simulink model "AGV_IFOC_BLOCKS"  (R2025a)
settings: Solver=ode4  StartTime=0.0  StopTime=t_stop_agv  FixedStep=h_step_agv  RelTol=1e-3
InitFcn:
  | addpath(fileparts(get_param('AGV_IFOC_BLOCKS','FileName'))); bm_drive = 'IFOC'; bm_model = 'AGV_IFOC_BLOCKS'; block_model_params;
values from neighbouring files (symbols this model uses):
  agv_fault_side_default = a.fault_side    [block_model_params.m]
  agv_fault_type_default = a.fault_type    [block_model_params.m]
  Bm = m.B    [block_model_params.m]
  Crr = a.Crr    [block_model_params.m]
  Esw = P.inv.Esw    [block_model_params.m]
  eta_g = a.eta_g    [block_model_params.m]
  flux_mode_default = c.flux_mode    [block_model_params.m]
  G_gear = a.G    [block_model_params.m]
  h_step_agv = 25e-6    (= 2.5e-05)    [block_model_params.m]
  Iref_sw = P.inv.Iref    [block_model_params.m]
  Jm = m.J    [block_model_params.m]
  ke = m.ke    [block_model_params.m]
  kh = m.kh    [block_model_params.m]
  Ki_i = c.Ki_i    [block_model_params.m]
  Ko = c.Ko    [block_model_params.m]
  Kp_i = c.Kp_i    [block_model_params.m]
  Kp_w = c.Kp_w    [block_model_params.m]
  L_look = a.L_look    [block_model_params.m]
  Llr = m.Llr    [block_model_params.m]
  Lls = m.Lls    [block_model_params.m]
  Lm0 = m.Lm0    [block_model_params.m]
  Lm_rated = m.Lm_rated    [block_model_params.m]
  lut_an = P.lut.psi    [block_model_params.m]
  lut_ml = bm_P.lut.psi; end    [block_model_params.m]
  lut_T = P.lut.T(:)'    [block_model_params.m]
  lut_w = P.lut.w(:)'    [block_model_params.m]
  Lx = a.Lx    [block_model_params.m]
  Ly = a.Ly    [block_model_params.m]
  m_payload = a.m_payload    [block_model_params.m]
  m_robot = a.m_robot    [block_model_params.m]
  mlp_b1 = double(bm_M.b1(:))    [block_model_params.m]
  mlp_b2 = double(bm_M.b2)    [block_model_params.m]
  mlp_W1 = double(bm_M.W1)    [block_model_params.m]
  mlp_W2 = double(bm_M.W2(:)')    [block_model_params.m]
  mlp_x_mu = double(bm_M.x_mu(:))    [block_model_params.m]
  mlp_x_sd = double(bm_M.x_sd(:))    [block_model_params.m]
  mlp_y_mu = double(bm_M.y_mu)    [block_model_params.m]
  mlp_y_sd = double(bm_M.y_sd)    [block_model_params.m]
  mras_Ki = c.mras_Ki    [block_model_params.m]
  mras_Kp = c.mras_Kp    [block_model_params.m]
  mras_wc = c.mras_wc    [block_model_params.m]
  NT_agv = max(1, round(Ts/h_step_agv))    [block_model_params.m]
  pp = m.p    [block_model_params.m]
  psi_k = m.psi_k    [block_model_params.m]
  r_wheel = a.r_wheel    [block_model_params.m]
  rce = P.inv.rce    [block_model_params.m]
  Rr = m.Rr    [block_model_params.m]
  Rs = m.Rs    [block_model_params.m]
  s32 = sqrt(3)/2    [block_model_params.m]
  sat_a = m.sat_a    [block_model_params.m]
  sat_b = m.sat_b    [block_model_params.m]
  sat_on = m.sat_on    [block_model_params.m]
  Te_max = c.Te_max    [block_model_params.m]
  Ts = P.ctrl.Ts    [block_log_to_thesis.m]    (also in block_model_params.m = c.Ts)
  twopi = 2*pi    (= 6.28318530718)    [block_model_params.m]
  Vce0 = P.inv.Vce0    [block_model_params.m]
  Vdc = P.inv.Vdc    [block_model_params.m]
  Vref_sw = P.inv.Vref    [block_model_params.m]
  W_track = a.W_track    [block_model_params.m]
(part 2 of 4)

== system AGV_IFOC_BLOCKS/Right wheel drive/Controller ==
  ia_m : Inport
  ib_m : Inport  Port=2
  ic_m : Inport  Port=3
  w_m : Inport  Port=4
  w_ref : Inport  Port=5
  flux_sel : Inport  Port=6
  lut_sel : Inport  Port=7
  speed_mode : Inport  Port=8
  Applied voltage and current observer : Subsystem
  Current reconstruction : Subsystem
  Fault detection and isolation : Subsystem
  Flux reference : Subsystem
  IFOC current control and SVPWM : Subsystem
  MRAS speed estimator : Subsystem
  Model inductances : Subsystem
  Speed controller : Subsystem
  Te_est not used in IFOC : Constant  Value=0
  ia_m sample : ZeroOrderHold  SampleTime=Ts
  ib_m sample : ZeroOrderHold  SampleTime=Ts
  ic_m sample : ZeroOrderHold  SampleTime=Ts
  w_m sample : ZeroOrderHold  SampleTime=Ts
  w_ref sample : ZeroOrderHold  SampleTime=Ts
  da out : Outport
  db out : Outport  Port=2
  dc out : Outport  Port=3
  neutral out : Outport  Port=4
  w_u out : Outport  Port=5
  w_est out : Outport  Port=6
  Te_ref out : Outport  Port=7
  psi_ref out : Outport  Port=8
  psi_est out : Outport  Port=9
  Te_est out : Outport  Port=10
  f_speed out : Outport  Port=11
  f_cur out : Outport  Port=12
  f_open out : Outport  Port=13
  wires:
  ia_m/1 -> ia_m sample/1
  ib_m/1 -> ib_m sample/1
  ic_m/1 -> ic_m sample/1
  w_m/1 -> w_m sample/1
  w_ref/1 -> w_ref sample/1
  Flux reference/3(psi_ref_p out) -> Model inductances/1(psi_ref_p)
  ia_m sample/1 -> Current reconstruction/1(ia_m), Fault detection and isolation/2(ia_m)
  ib_m sample/1 -> Current reconstruction/2(ib_m), Fault detection and isolation/3(ib_m), Applied voltage and current observer/4(ib_m)
  ic_m sample/1 -> Current reconstruction/3(ic_m), Fault detection and isolation/4(ic_m)
  Fault detection and isolation/8(f_cur_p out) -> Current reconstruction/4(f_cur_p)
  Fault detection and isolation/9(neutral_p out) -> Current reconstruction/5(neutral_p)
  Applied voltage and current observer/3(obs1_p out) -> Current reconstruction/6(obs1_p)
  Applied voltage and current observer/4(obs3_p out) -> Current reconstruction/7(obs3_p)
  Model inductances/1(Lm_c out) -> Current reconstruction/8(Lm_c), MRAS speed estimator/7(Lm_c), IFOC current control and SVPWM/8(Lm_c), Applied voltage and current observer/6(Lm_c)
  Model inductances/3(Lr_c out) -> Current reconstruction/9(Lr_c), MRAS speed estimator/8(Lr_c), IFOC current control and SVPWM/9(Lr_c), Applied voltage and current observer/8(Lr_c)
  Model inductances/6(D_c out) -> Current reconstruction/10(D_c), Applied voltage and current observer/9(D_c)
  Current reconstruction/1(i_alpha out) -> MRAS speed estimator/1(i_alpha), IFOC current control and SVPWM/1(i_alpha)
  Current reconstruction/2(i_beta out) -> MRAS speed estimator/2(i_beta), IFOC current control and SVPWM/2(i_beta)
  Current reconstruction/4(i_alpha_p out) -> MRAS speed estimator/3(i_alpha_p)
  Current reconstruction/5(i_beta_p out) -> MRAS speed estimator/4(i_beta_p)
  Applied voltage and current observer/1(va_app_p out) -> MRAS speed estimator/5(va_app_p)
  Applied voltage and current observer/2(vb_app_p out) -> MRAS speed estimator/6(vb_app_p)
  Model inductances/4(sLs_c out) -> MRAS speed estimator/9(sLs_c), IFOC current control and SVPWM/10(sLs_c)
  Model inductances/5(tr_c out) -> MRAS speed estimator/10(tr_c), IFOC current control and SVPWM/11(tr_c)
  w_ref sample/1 -> MRAS speed estimator/11(w_ref), Fault detection and isolation/5(w_ref), Speed controller/1(w_ref)
  w_m sample/1 -> MRAS speed estimator/12(w_m), Fault detection and isolation/1(w_m)
  Fault detection and isolation/7(f_speed_p out) -> MRAS speed estimator/13(f_speed_p)
  Flux reference/4(trans_t_p out) -> MRAS speed estimator/14(trans_t_p)
  Flux reference/5(dpsi_rate_p out) -> MRAS speed estimator/15(dpsi_p)
  Speed controller/3(Te_ref_p out) -> MRAS speed estimator/16(Te_ref_p)
  Fault detection and isolation/10(Te_lim_p out) -> MRAS speed estimator/17(Te_lim_p)
  MRAS speed estimator/1(w_est out) -> Fault detection and isolation/6(w_est), w_est out/1
  MRAS speed estimator/2(mras_ok out) -> Fault detection and isolation/7(mras_ok)
  Current reconstruction/3(ia_hat out) -> Fault detection and isolation/8(ia_hat)
  Fault detection and isolation/6(w_u out) -> Speed controller/2(w_u), Flux reference/3(w_u), IFOC current control and SVPWM/6(w_u), Applied voltage and current observer/5(w_u), w_u out/1
  Fault detection and isolation/5(Te_lim out) -> Speed controller/3(Te_lim)
  speed_mode/1 -> Speed controller/4(mode)
  Speed controller/2(e_w out) -> Flux reference/1(e_w)
  Speed controller/1(Te_ref out) -> Flux reference/2(Te_ref), IFOC current control and SVPWM/5(Te_ref), Te_ref out/1
  flux_sel/1 -> Flux reference/4(flux_sel)
  lut_sel/1 -> Flux reference/5(lut_sel)
  Flux reference/1(psi_ref out) -> IFOC current control and SVPWM/3(psi_ref), psi_ref out/1
  Flux reference/2(dpsi_rate out) -> IFOC current control and SVPWM/4(dpsi_rate)
  Fault detection and isolation/4(neutral out) -> IFOC current control and SVPWM/7(neutral), neutral out/1
  Te_est not used in IFOC/1 -> Te_est out/1
  IFOC current control and SVPWM/1(da out) -> Applied voltage and current observer/1(da), da out/1
  IFOC current control and SVPWM/2(db out) -> Applied voltage and current observer/2(db), db out/1
  IFOC current control and SVPWM/3(dc out) -> Applied voltage and current observer/3(dc), dc out/1
  Model inductances/2(Ls_c out) -> Applied voltage and current observer/7(Ls_c)
  IFOC current control and SVPWM/4(psir_est out) -> psi_est out/1
  Fault detection and isolation/1(f_speed out) -> f_speed out/1
  Fault detection and isolation/2(f_cur out) -> f_cur out/1
  Fault detection and isolation/3(f_open out) -> f_open out/1

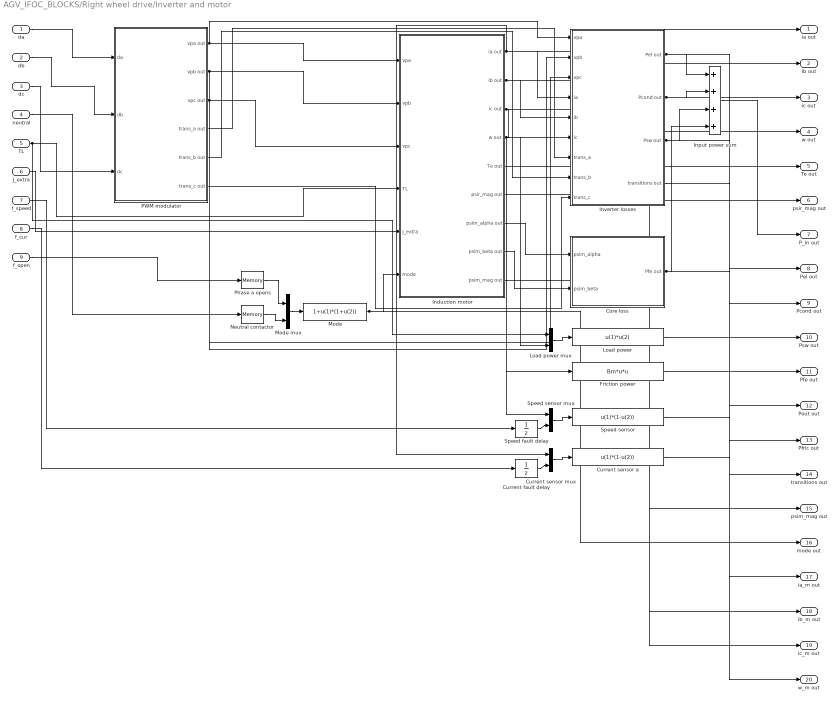
== system AGV_IFOC_BLOCKS/Right wheel drive/Inverter and motor ==
  da : Inport
  db : Inport  Port=2
  dc : Inport  Port=3
  neutral : Inport  Port=4
  TL : Inport  Port=5
  J_extra : Inport  Port=6
  f_speed : Inport  Port=7
  f_cur : Inport  Port=8
  f_open : Inport  Port=9
  Core loss : Subsystem
  Current fault delay : UnitDelay  SampleTime=Ts  HasFrameUpgradeWarning=on
  Current sensor a : Fcn  Expr=u(1)*(1-u(2))
  Current sensor mux : Mux  Inputs=2
  Friction power : Fcn  Expr=Bm*u*u
  Induction motor : Subsystem
  Input power sum : Sum  Inputs=++++
  Inverter losses : Subsystem
  Load power : Fcn  Expr=u(1)*u(2)
  Load power mux : Mux  Inputs=2
  Mode : Fcn  Expr=1+u(1)*(1+u(2))
  Mode mux : Mux  Inputs=2
  Neutral contactor : Memory
  PWM modulator : Subsystem
  Phase a opens : Memory
  Speed fault delay : UnitDelay  SampleTime=Ts  HasFrameUpgradeWarning=on
  Speed sensor : Fcn  Expr=u(1)*(1-u(2))
  Speed sensor mux : Mux  Inputs=2
  ia out : Outport
  ib out : Outport  Port=2
  ic out : Outport  Port=3
  w out : Outport  Port=4
  Te out : Outport  Port=5
  psir_mag out : Outport  Port=6
  P_in out : Outport  Port=7
  Pel out : Outport  Port=8
  Pcond out : Outport  Port=9
  Psw out : Outport  Port=10
  Pfe out : Outport  Port=11
  Pout out : Outport  Port=12
  Pfric out : Outport  Port=13
  transitions out : Outport  Port=14
  psim_mag out : Outport  Port=15
  mode out : Outport  Port=16
  ia_m out : Outport  Port=17
  ib_m out : Outport  Port=18
  ic_m out : Outport  Port=19
  w_m out : Outport  Port=20
  wires:
  neutral/1 -> Neutral contactor/1
  f_open/1 -> Phase a opens/1
  Phase a opens/1 -> Mode mux/1
  Neutral contactor/1 -> Mode mux/2
  Mode mux/1 -> Mode/1
  da/1 -> PWM modulator/1(da)
  db/1 -> PWM modulator/2(db)
  dc/1 -> PWM modulator/3(dc)
  PWM modulator/1(vpa out) -> Induction motor/1(vpa), Inverter losses/1(vpa)
  PWM modulator/2(vpb out) -> Induction motor/2(vpb), Inverter losses/2(vpb)
  PWM modulator/3(vpc out) -> Induction motor/3(vpc), Inverter losses/3(vpc)
  TL/1 -> Induction motor/4(TL), Load power mux/1
  J_extra/1 -> Induction motor/5(J_extra)
  Mode/1 -> Induction motor/6(mode), mode out/1
  Induction motor/1(ia out) -> Inverter losses/4(ia), Current sensor mux/1, ia out/1
  PWM modulator/4(trans_a out) -> Inverter losses/7(trans_a)
  Induction motor/2(ib out) -> Inverter losses/5(ib), ib out/1, ib_m out/1
  PWM modulator/5(trans_b out) -> Inverter losses/8(trans_b)
  Induction motor/3(ic out) -> Inverter losses/6(ic), ic out/1, ic_m out/1
  PWM modulator/6(trans_c out) -> Inverter losses/9(trans_c)
  Induction motor/7(psim_alpha out) -> Core loss/1(psim_alpha)
  Induction motor/8(psim_beta out) -> Core loss/2(psim_beta)
  Induction motor/4(w out) -> Load power mux/2, Friction power/1, Speed sensor mux/1, w out/1
  Load power mux/1 -> Load power/1
  Inverter losses/1(Pel out) -> Input power sum/1, Pel out/1
  Inverter losses/2(Pcond out) -> Input power sum/2, Pcond out/1
  Inverter losses/3(Psw out) -> Input power sum/3, Psw out/1
  Core loss/1(Pfe out) -> Input power sum/4, Pfe out/1
  f_speed/1 -> Speed fault delay/1
  f_cur/1 -> Current fault delay/1
  Speed fault delay/1 -> Speed sensor mux/2
  Speed sensor mux/1 -> Speed sensor/1
  Current fault delay/1 -> Current sensor mux/2
  Current sensor mux/1 -> Current sensor a/1
  Induction motor/5(Te out) -> Te out/1
  Induction motor/6(psir_mag out) -> psir_mag out/1
  Input power sum/1 -> P_in out/1
  Load power/1 -> Pout out/1
  Friction power/1 -> Pfric out/1
  Inverter losses/4(transitions out) -> transitions out/1
  Induction motor/9(psim_mag out) -> psim_mag out/1
  Current sensor a/1 -> ia_m out/1
  Speed sensor/1 -> w_m out/1

== system AGV_IFOC_BLOCKS/Left wheel drive/Controller/Applied voltage and current observer ==
  da : Inport
  db : Inport  Port=2
  dc : Inport  Port=3
  ib_m : Inport  Port=4
  w_u : Inport  Port=5
  Lm_c : Inport  Port=6
  Ls_c : Inport  Port=7
  Lr_c : Inport  Port=8
  D_c : Inport  Port=9
  ib error : Fcn  Expr=u(1)-(-0.5*u(2)+s32*u(3))
  ib error in : Mux  Inputs=3
  obs ir_alpha : Fcn  Expr=(u(6)*u(3)-u(5)*u(1))/u(8)
  obs ir_alpha in : Mux  Inputs=8
  obs ir_beta : Fcn  Expr=(u(6)*u(4)-u(5)*u(2))/u(8)
  obs ir_beta in : Mux  Inputs=8
  obs is_alpha : Fcn  Expr=(u(7)*u(1)-u(5)*u(3))/u(8)
  obs is_alpha in : Mux  Inputs=8
  obs is_beta : Fcn  Expr=(u(7)*u(2)-u(5)*u(4))/u(8)
  obs is_beta in : Mux  Inputs=8
  obs1 : Fcn  Expr=u(1)+Ts*(u(2)-Rs*u(3)+Ko*(-0.5)*u(4))
  obs1 in : Mux
  obs1(k-1) : UnitDelay  SampleTime=Ts  HasFrameUpgradeWarning=on
  obs2 : Fcn  Expr=u(1)+Ts*(u(2)-Rs*u(3)+Ko*s32*u(4))
  obs2 in : Mux
  obs2(k-1) : UnitDelay  SampleTime=Ts  HasFrameUpgradeWarning=on
  obs3 : Fcn  Expr=u(1)+Ts*(-Rr*u(3)-pp*u(4)*u(2))
  obs3 in : Mux
  obs3(k-1) : UnitDelay  SampleTime=Ts  HasFrameUpgradeWarning=on
  obs4 : Fcn  Expr=u(2)+Ts*(-Rr*u(3)+pp*u(4)*u(1))
  obs4 in : Mux
  obs4(k-1) : UnitDelay  SampleTime=Ts  HasFrameUpgradeWarning=on
  va_app : Fcn  Expr=(2/3)*((u(1)-0.5)*Vdc-0.5*((u(2)-0.5)*Vdc+(u(3)-0.5)*Vdc))
  va_app in : Mux  Inputs=3
  va_app(k-1) : UnitDelay  SampleTime=Ts  HasFrameUpgradeWarning=on
  vb_app : Fcn  Expr=((u(1)-0.5)*Vdc-(u(2)-0.5)*Vdc)/sqrt(3)
  vb_app in : Mux  Inputs=2
  vb_app(k-1) : UnitDelay  SampleTime=Ts  HasFrameUpgradeWarning=on
  va_app_p out : Outport
  vb_app_p out : Outport  Port=2
  obs1_p out : Outport  Port=3
  obs3_p out : Outport  Port=4
  wires:
  da/1 -> va_app in/1
  db/1 -> va_app in/2, vb_app in/1
  dc/1 -> va_app in/3, vb_app in/2
  va_app in/1 -> va_app/1
  va_app/1 -> va_app(k-1)/1, obs1 in/2
  vb_app in/1 -> vb_app/1
  vb_app/1 -> vb_app(k-1)/1, obs2 in/2
  obs1(k-1)/1 -> obs is_alpha in/1, obs is_beta in/1, obs ir_alpha in/1, obs ir_beta in/1, obs1 in/1, obs1_p out/1
  obs2(k-1)/1 -> obs is_alpha in/2, obs is_beta in/2, obs ir_alpha in/2, obs ir_beta in/2, obs2 in/1
  obs3(k-1)/1 -> obs is_alpha in/3, obs is_beta in/3, obs ir_alpha in/3, obs ir_beta in/3, obs3 in/1, obs4 in/1, obs3_p out/1
  obs4(k-1)/1 -> obs is_alpha in/4, obs is_beta in/4, obs ir_alpha in/4, obs ir_beta in/4, obs3 in/2, obs4 in/2
  Lm_c/1 -> obs is_alpha in/5, obs is_beta in/5, obs ir_alpha in/5, obs ir_beta in/5
  Ls_c/1 -> obs is_alpha in/6, obs is_beta in/6, obs ir_alpha in/6, obs ir_beta in/6
  Lr_c/1 -> obs is_alpha in/7, obs is_beta in/7, obs ir_alpha in/7, obs ir_beta in/7
  D_c/1 -> obs is_alpha in/8, obs is_beta in/8, obs ir_alpha in/8, obs ir_beta in/8
  obs is_alpha in/1 -> obs is_alpha/1
  obs is_beta in/1 -> obs is_beta/1
  obs ir_alpha in/1 -> obs ir_alpha/1
  obs ir_beta in/1 -> obs ir_beta/1
  ib_m/1 -> ib error in/1
  obs is_alpha/1 -> ib error in/2, obs1 in/3
  obs is_beta/1 -> ib error in/3, obs2 in/3
  ib error in/1 -> ib error/1
  ib error/1 -> obs1 in/4, obs2 in/4
  obs1 in/1 -> obs1/1
  obs1/1 -> obs1(k-1)/1
  obs2 in/1 -> obs2/1
  obs2/1 -> obs2(k-1)/1
  obs ir_alpha/1 -> obs3 in/3
  w_u/1 -> obs3 in/4, obs4 in/4
  obs3 in/1 -> obs3/1
  obs3/1 -> obs3(k-1)/1
  obs ir_beta/1 -> obs4 in/3
  obs4 in/1 -> obs4/1
  obs4/1 -> obs4(k-1)/1
  va_app(k-1)/1 -> va_app_p out/1
  vb_app(k-1)/1 -> vb_app_p out/1

== system AGV_IFOC_BLOCKS/Left wheel drive/Controller/Current reconstruction ==
  ia_m : Inport
  ib_m : Inport  Port=2
  ic_m : Inport  Port=3
  f_cur_p : Inport  Port=4
  neutral_p : Inport  Port=5
  obs1_p : Inport  Port=6
  obs3_p : Inport  Port=7
  Lm_c : Inport  Port=8
  Lr_c : Inport  Port=9
  D_c : Inport  Port=10
  i_alpha : Fcn  Expr=((u(1)>0.5)*(-(u(2)+u(3))/3)+(1-(u(1)>0.5))*(u(4)))
  i_alpha in : Mux
  i_alpha(k-1) : UnitDelay  SampleTime=Ts  HasFrameUpgradeWarning=on
  i_beta : Fcn  Expr=((u(1)>0.5)*((u(2)-u(3))/sqrt(3))+(1-(u(1)>0.5))*((u(4)+2*u(2))/sqrt(3)))
  i_beta in : Mux
  i_beta(k-1) : UnitDelay  SampleTime=Ts  HasFrameUpgradeWarning=on
  ia_hat : Fcn  Expr=(u(1)*u(3)-u(2)*u(4))/u(5)
  ia_hat in : Mux  Inputs=5
  ia_u : Fcn  Expr=((u(1)>0.5)*(u(2))+(1-(u(1)>0.5))*(u(3)))
  ia_u in : Mux  Inputs=3
  i_alpha out : Outport
  i_beta out : Outport  Port=2
  ia_hat out : Outport  Port=3
  i_alpha_p out : Outport  Port=4
  i_beta_p out : Outport  Port=5
  wires:
  Lr_c/1 -> ia_hat in/1
  Lm_c/1 -> ia_hat in/2
  obs1_p/1 -> ia_hat in/3
  obs3_p/1 -> ia_hat in/4
  D_c/1 -> ia_hat in/5
  ia_hat in/1 -> ia_hat/1
  f_cur_p/1 -> ia_u in/1
  ia_hat/1 -> ia_u in/2, ia_hat out/1
  ia_m/1 -> ia_u in/3
  ia_u in/1 -> ia_u/1
  neutral_p/1 -> i_alpha in/1, i_beta in/1
  ib_m/1 -> i_alpha in/2, i_beta in/2
  ic_m/1 -> i_alpha in/3, i_beta in/3
  ia_u/1 -> i_alpha in/4, i_beta in/4
  i_alpha in/1 -> i_alpha/1
  i_alpha/1 -> i_alpha(k-1)/1, i_alpha out/1
  i_beta in/1 -> i_beta/1
  i_beta/1 -> i_beta(k-1)/1, i_beta out/1
  i_alpha(k-1)/1 -> i_alpha_p out/1
  i_beta(k-1)/1 -> i_beta_p out/1

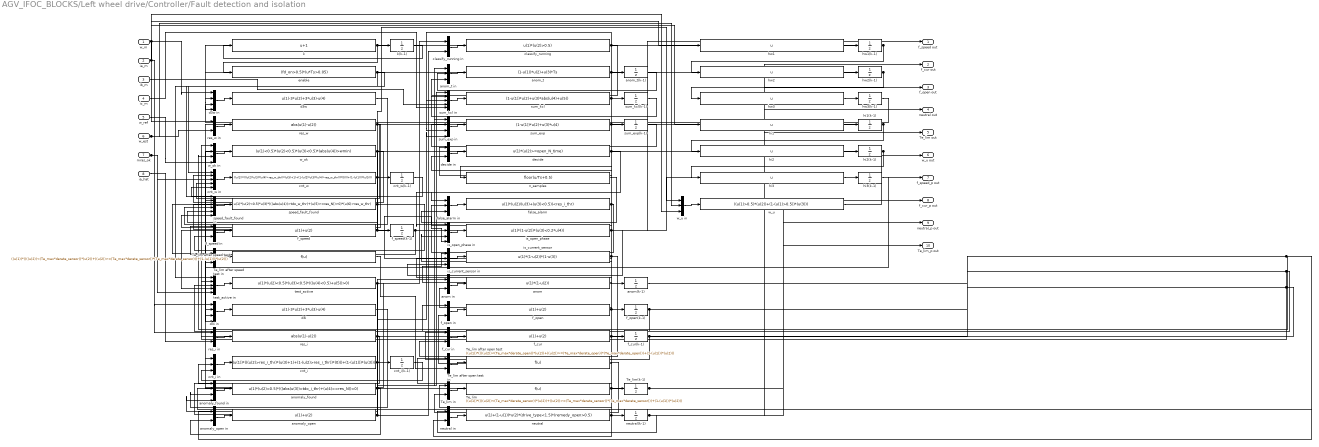
== system AGV_IFOC_BLOCKS/Left wheel drive/Controller/Fault detection and isolation ==
  w_m : Inport
  ia_m : Inport  Port=2
  ib_m : Inport  Port=3
  ic_m : Inport  Port=4
  w_ref : Inport  Port=5
  w_est : Inport  Port=6
  mras_ok : Inport  Port=7
  ia_hat : Inport  Port=8
  Te_lim : Fcn  Expr=((u(1))*((((u(2))<(Te_max*derate_sensor))*(u(2))+((u(2))>=(Te_max*derate_sensor))*(Te_max*derate_sensor)))+(1-(u(1)))*(u(2)))
  Te_lim after open test : Fcn  Expr=((u(1))*((((u(2))<(Te_max*derate_open))*(u(2))+((u(2))>=(Te_max*derate_open))*(Te_max*derate_open)))+(1-(u(1)))*(u(2)))
  Te_lim after open test in : Mux  Inputs=2
  Te_lim after speed test : Fcn  Expr=((u(1))*((((u(2))<(Te_max*derate_sensor))*(u(2))+((u(2))>=(Te_max*derate_sensor))*(Te_max*derate_sensor)))+(1-(u(1)))*(u(2)))
  Te_lim after speed test in : Mux  Inputs=2
  Te_lim in : Mux  Inputs=2
  Te_lim(k-1) : UnitDelay  InitialCondition=Te_max  SampleTime=Ts  HasFrameUpgradeWarning=on
  anom : Fcn  Expr=u(1)*(1-u(2))
  anom in : Mux  Inputs=2
  anom(k-1) : UnitDelay  SampleTime=Ts  HasFrameUpgradeWarning=on
  anom_t : Fcn  Expr=(1-u(1))*u(2)+u(3)*Ts
  anom_t in : Mux  Inputs=3
  anom_t(k-1) : UnitDelay  SampleTime=Ts  HasFrameUpgradeWarning=on
  anomaly_found : Fcn  Expr=u(1)*(u(2)<0.5)*(((abs(u(3))>tdo_i_thr)+(u(4)>=res_N))>0)
  anomaly_found in : Mux
  anomaly_open : Fcn  Expr=u(1)+u(2)
  anomaly_open in : Mux  Inputs=2
  classify_running : Fcn  Expr=u(1)*(u(2)>0.5)
  classify_running in : Mux  Inputs=2
  cnt_i : Fcn  Expr=((u(1))*(((u(2)>res_i_thr)*(u(3)+1)+(1-(u(2)>res_i_thr))*(0)))+(1-(u(1)))*(u(3)))
  cnt_i in : Mux  Inputs=3
  cnt_i(k-1) : UnitDelay  SampleTime=Ts  HasFrameUpgradeWarning=on
  cnt_w : Fcn  Expr=((u(1))*(((u(2)*u(3)*(u(4)>res_w_thr))*(u(5)+1)+(1-(u(2)*u(3)*(u(4)>res_w_thr)))*(0)))+(1-(u(1)))*(u(5)))
  cnt_w in : Mux  Inputs=5
  cnt_w(k-1) : UnitDelay  SampleTime=Ts  HasFrameUpgradeWarning=on
  d3i : Fcn  Expr=u(1)-3*u(2)+3*u(3)-u(4)
  d3i in : Mux
  d3w : Fcn  Expr=u(1)-3*u(2)+3*u(3)-u(4)
  d3w in : Mux
  decide : Fcn  Expr=u(1)*(u(2)>=open_N_time)
  decide in : Mux  Inputs=2
  enable : Fcn  Expr=(fd_on>0.5)*(u*Ts>0.05)
  f_cur : Fcn  Expr=u(1)+u(2)
  f_cur in : Mux  Inputs=2
  f_cur(k-1) : UnitDelay  SampleTime=Ts  HasFrameUpgradeWarning=on
  f_open : Fcn  Expr=u(1)+u(2)
  f_open in : Mux  Inputs=2
  f_open(k-1) : UnitDelay  SampleTime=Ts  HasFrameUpgradeWarning=on
  f_speed : Fcn  Expr=u(1)+u(2)
  f_speed in : Mux  Inputs=2
  f_speed(k-1) : UnitDelay  SampleTime=Ts  HasFrameUpgradeWarning=on
  false_alarm : Fcn  Expr=u(1)*(u(2)/(u(3)+(u(3)<0.5))<res_i_thr)
  false_alarm in : Mux  Inputs=3
  hi1 : Fcn  Expr=u
  hi1(k-1) : UnitDelay  SampleTime=Ts  HasFrameUpgradeWarning=on
  hi2 : Fcn  Expr=u
  hi2(k-1) : UnitDelay  SampleTime=Ts  HasFrameUpgradeWarning=on
  hi3 : Fcn  Expr=u
  hi3(k-1) : UnitDelay  SampleTime=Ts  HasFrameUpgradeWarning=on
  hw1 : Fcn  Expr=u
  hw1(k-1) : UnitDelay  SampleTime=Ts  HasFrameUpgradeWarning=on
  hw2 : Fcn  Expr=u
  hw2(k-1) : UnitDelay  SampleTime=Ts  HasFrameUpgradeWarning=on
  hw3 : Fcn  Expr=u
  hw3(k-1) : UnitDelay  SampleTime=Ts  HasFrameUpgradeWarning=on
  is_current_sensor : Fcn  Expr=u(1)*(1-u(2))*(1-u(3))
  is_current_sensor in : Mux  Inputs=3
  is_open_phase : Fcn  Expr=u(1)*(1-u(2))*(u(3)<0.2*u(4))
  is_open_phase in : Mux
  k : Fcn  Expr=u+1
  k(k-1) : UnitDelay  SampleTime=Ts  HasFrameUpgradeWarning=on
  n_samples : Fcn  Expr=floor(u/Ts+0.5)
  neutral : Fcn  Expr=u(1)+(1-u(1))*u(2)*(drive_type<1.5)*(remedy_open>0.5)
  neutral in : Mux  Inputs=2
  neutral(k-1) : UnitDelay  SampleTime=Ts  HasFrameUpgradeWarning=on
  res_i : Fcn  Expr=abs(u(1)-u(2))
  res_i in : Mux  Inputs=2
  res_w : Fcn  Expr=abs(u(1)-u(2))
  res_w in : Mux  Inputs=2
  speed_fault_found : Fcn  Expr=u(1)*(u(2)<0.5)*u(3)*(((abs(u(4))>tdo_w_thr)+(u(5)>=res_N))>0)*(u(6)>res_w_thr)
  speed_fault_found in : Mux  Inputs=6
  sum_exp : Fcn  Expr=(1-u(1))*u(2)+u(3)*u(4)
  sum_exp in : Mux
  sum_exp(k-1) : UnitDelay  SampleTime=Ts  HasFrameUpgradeWarning=on
  sum_kcl : Fcn  Expr=(1-u(1))*u(2)+u(3)*abs(u(4)+u(5))
  sum_kcl in : Mux  Inputs=5
  sum_kcl(k-1) : UnitDelay  SampleTime=Ts  HasFrameUpgradeWarning=on
  test_active : Fcn  Expr=u(1)*(u(2)<0.5)*(u(3)<0.5)*(((u(4)<0.5)+u(5))>0)
  test_active in : Mux  Inputs=5
  w_ok : Fcn  Expr=(u(1)<0.5)*(u(2)<0.5)*(u(3)<0.5)*(abs(u(4))>wmin)
  w_ok in : Mux
  w_u : Fcn  Expr=((u(1)>0.5)*(u(2))+(1-(u(1)>0.5))*(u(3)))
  w_u in : Mux  Inputs=3
  f_speed out : Outport
  f_cur out : Outport  Port=2
  f_open out : Outport  Port=3
  neutral out : Outport  Port=4
  Te_lim out : Outport  Port=5
  w_u out : Outport  Port=6
  f_speed_p out : Outport  Port=7
  f_cur_p out : Outport  Port=8
  neutral_p out : Outport  Port=9
  Te_lim_p out : Outport  Port=10
  wires:
  k(k-1)/1 -> k/1
  k/1 -> k(k-1)/1, enable/1
  w_m/1 -> d3w in/1, res_w in/1, hw1/1, w_u in/3
  hw1(k-1)/1 -> d3w in/2, hw2/1
  hw2(k-1)/1 -> d3w in/3, hw3/1
  hw3(k-1)/1 -> d3w in/4
  d3w in/1 -> d3w/1
  w_est/1 -> res_w in/2, w_u in/2
  res_w in/1 -> res_w/1
  f_cur(k-1)/1 -> w_ok in/1, test_active in/2, f_cur in/1, f_cur_p out/1
  f_open(k-1)/1 -> w_ok in/2, test_active in/3, f_open in/1
  anom(k-1)/1 -> w_ok in/3, anomaly_found in/2, anomaly_open in/1
  w_ref/1 -> w_ok in/4
  w_ok in/1 -> w_ok/1
  enable/1 -> cnt_w in/1, speed_fault_found in/1, test_active in/1
  w_ok/1 -> cnt_w in/2, speed_fault_found in/3
  mras_ok/1 -> cnt_w in/3, test_active in/5
  res_w/1 -> cnt_w in/4, speed_fault_found in/6
  cnt_w(k-1)/1 -> cnt_w in/5
  cnt_w in/1 -> cnt_w/1
  cnt_w/1 -> cnt_w(k-1)/1, speed_fault_found in/5
  f_speed(k-1)/1 -> speed_fault_found in/2, f_speed in/1, f_speed_p out/1
  d3w/1 -> speed_fault_found in/4
  speed_fault_found in/1 -> speed_fault_found/1
  speed_fault_found/1 -> f_speed in/2, Te_lim after speed test in/1
  f_speed in/1 -> f_speed/1
  f_speed/1 -> f_speed(k-1)/1, test_active in/4, w_u in/1, f_speed out/1
  Te_lim(k-1)/1 -> Te_lim after speed test in/2, Te_lim_p out/1
  Te_lim after speed test in/1 -> Te_lim after speed test/1
  test_active in/1 -> test_active/1
  ia_m/1 -> d3i in/1, res_i in/1, hi1/1
  hi1(k-1)/1 -> d3i in/2, hi2/1
  hi2(k-1)/1 -> d3i in/3, hi3/1
  hi3(k-1)/1 -> d3i in/4
  d3i in/1 -> d3i/1
  ia_hat/1 -> res_i in/2
  res_i in/1 -> res_i/1
  test_active/1 -> cnt_i in/1, anomaly_found in/1, classify_running in/1
  res_i/1 -> cnt_i in/2, sum_exp in/4
  cnt_i(k-1)/1 -> cnt_i in/3
  cnt_i in/1 -> cnt_i/1
  cnt_i/1 -> cnt_i(k-1)/1, anomaly_found in/4
  d3i/1 -> anomaly_found in/3
  anomaly_found in/1 -> anomaly_found/1
  anomaly_found/1 -> anomaly_open in/2, anom_t in/1, sum_kcl in/1, sum_exp in/1
  anomaly_open in/1 -> anomaly_open/1
  anomaly_open/1 -> classify_running in/2, anom in/1
  classify_running in/1 -> classify_running/1
  anom_t(k-1)/1 -> anom_t in/2
  classify_running/1 -> anom_t in/3, sum_kcl in/3, sum_exp in/3, decide in/1
  anom_t in/1 -> anom_t/1
  anom_t/1 -> anom_t(k-1)/1, decide in/2, n_samples/1
  sum_kcl(k-1)/1 -> sum_kcl in/2
  ib_m/1 -> sum_kcl in/4
  ic_m/1 -> sum_kcl in/5
  sum_kcl in/1 -> sum_kcl/1
  sum_kcl/1 -> sum_kcl(k-1)/1, is_open_phase in/3
  sum_exp(k-1)/1 -> sum_exp in/2
  sum_exp in/1 -> sum_exp/1
  sum_exp/1 -> sum_exp(k-1)/1, false_alarm in/2, is_open_phase in/4
  decide in/1 -> decide/1
  decide/1 -> false_alarm in/1, is_open_phase in/1, is_current_sensor in/1, anom in/2
  n_samples/1 -> false_alarm in/3
  false_alarm in/1 -> false_alarm/1
  false_alarm/1 -> is_open_phase in/2, is_current_sensor in/2
  is_open_phase in/1 -> is_open_phase/1
  is_open_phase/1 -> is_current_sensor in/3, f_open in/2, Te_lim after open test in/1, neutral in/2
  is_current_sensor in/1 -> is_current_sensor/1
  anom in/1 -> anom/1
  anom/1 -> anom(k-1)/1
  f_open in/1 -> f_open/1
  f_open/1 -> f_open(k-1)/1, f_open out/1
  is_current_sensor/1 -> f_cur in/2, Te_lim in/1
  f_cur in/1 -> f_cur/1
  f_cur/1 -> f_cur(k-1)/1, f_cur out/1
  Te_lim after speed test/1 -> Te_lim after open test in/2
  Te_lim after open test in/1 -> Te_lim after open test/1
  Te_lim after open test/1 -> Te_lim in/2
  Te_lim in/1 -> Te_lim/1
  Te_lim/1 -> Te_lim(k-1)/1, Te_lim out/1
  neutral(k-1)/1 -> neutral in/1, neutral_p out/1
  neutral in/1 -> neutral/1
  neutral/1 -> neutral(k-1)/1, neutral out/1
  hw1/1 -> hw1(k-1)/1
  hw2/1 -> hw2(k-1)/1
  hw3/1 -> hw3(k-1)/1
  hi1/1 -> hi1(k-1)/1
  hi2/1 -> hi2(k-1)/1
  hi3/1 -> hi3(k-1)/1
  w_u in/1 -> w_u/1
  w_u/1 -> w_u out/1

== system AGV_IFOC_BLOCKS/Left wheel drive/Controller/Flux reference ==
  e_w : Inport
  Te_ref : Inport  Port=2
  w_u : Inport  Port=3
  flux_sel : Inport  Port=4
  lut_sel : Inport  Port=5
  LUT ML : Lookup_n-D  BreakpointsForDimension1=lut_w  BreakpointsForDimension2=lut_T  Table=lut_ml  ExtrapMethod=Clip  InternalRulePriority=Speed  RndMeth=Simplest
      settings: InputPortMap=u0,u1
  LUT analytic : Lookup_n-D  BreakpointsForDimension1=lut_w  BreakpointsForDimension2=lut_T  Table=lut_an  ExtrapMethod=Clip  InternalRulePriority=Speed  RndMeth=Simplest
      settings: InputPortMap=u0,u1
  LUT select : MultiPortSwitch  Inputs=2  SaturateOnIntegerOverflow=off  InputSameDT=off
  MLP network : Subsystem
  Te_ref_f : Fcn  Expr=u(1)+Ts/0.05*(u(2)-u(1))
  Te_ref_f in : Mux  Inputs=2
  Te_ref_f(k-1) : UnitDelay  SampleTime=Ts  HasFrameUpgradeWarning=on
  abs Te_ref_f : Fcn  Expr=abs(u)
  abs w_u : Fcn  Expr=abs(u)
  dpsi : Fcn  Expr=((((((u(1)-u(2))>(-psi_rate*Ts))*(u(1)-u(2))+((u(1)-u(2))<=(-psi_rate*Ts))*(-psi_rate*Ts)))<(psi_rate*Ts))*((((u(1)-u(2))>(-psi_rate*Ts))*(u(1)-u(2))+((u(1)-u(2))<=(-psi_rate*Ts))*(-psi_rate*Ts)))+(((((u(1)-u(2))>(-psi_rate*Ts))*(u(1)-u(2))+((u(1)-u(2))<=(-psi_rate*Ts))*(-psi_rate*Ts)))>=(psi_rate*Ts))*(psi_rate*Ts))
  dpsi in : Mux  Inputs=2
  dpsi_rate : Fcn  Expr=u/Ts
  dpsi_rate(k-1) : UnitDelay  SampleTime=Ts  HasFrameUpgradeWarning=on
  psi_ref : Fcn  Expr=u(1)+u(2)
  psi_ref in : Mux  Inputs=2
  psi_ref(k-1) : UnitDelay  SampleTime=Ts  HasFrameUpgradeWarning=on
  psi_target : Fcn  Expr=((u(1)>0)*(psi_r_rated)+(1-(u(1)>0))*(((((((((u(2)<1.5)*(psi_r_rated)+(1-(u(2)<1.5))*(((u(2)<2.5)*(psi_fixed)+(1-(u(2)<2.5))*(((u(2)<3.5)*(u(3))+(1-(u(2)<3.5))*(u(4))))))))>(psi_min))*(((u(2)<1.5)*(psi_r_rated)+(1-(u(2)<1.5))*(((u(2)<2.5)*(psi_fixed)+(1-(u(2)<2.5))*(((u(2)<3.5)*(u(3))+(1-(u(2)<3.5))*(u(4))))))))+((((u(2)<1.5)*(psi_r_rated)+(1-(u(2)<1.5))*(((u(2)<2.5)*(psi_fixed)+(1-(u(2)<2.5))*(((u(2)<3.5)*(u(3))+(1-(u(2)<3.5))*(u(4))))))))<=(psi_min))*(psi_min)))<(psi_r_rated))*((((((u(2)<1.5)*(psi_r_rated)+(1-(u(2)<1.5))*(((u(2)<2.5)*(psi_fixed)+(1-(u(2)<2.5))*(((u(2)<3.5)*(u(3))+(1-(u(2)<3.5))*(u(4))))))))>(psi_min))*(((u(2)<1.5)*(psi_r_rated)+(1-(u(2)<1.5))*(((u(2)<2.5)*(psi_fixed)+(1-(u(2)<2.5))*(((u(2)<3.5)*(u(3))+(1-(u(2)<3.5))*(u(4))))))))+((((u(2)<1.5)*(psi_r_rated)+(1-(u(2)<1.5))*(((u(2)<2.5)*(psi_fixed)+(1-(u(2)<2.5))*(((u(2)<3.5)*(u(3))+(1-(u(2)<3.5))*(u(4))))))))<=(psi_min))*(psi_min)))+(((((((u(2)<1.5)*(psi_r_rated)+(1-(u(2)<1.5))*(((u(2)<2.5)*(psi_fixed)+(1-(u(2)<2.5))*(((u(2)<3.5)*(u(3))+(1-(u(2)<3.5))*(u(4))))))))>(psi_min))*(((u(2)<1.5)*(psi_r_rated)+(1-(u(2)<1.5))*(((u(2)<2.5)*(psi_fixed)+(1-(u(2)<2.5))*(((u(2)<3.5)*(u(3))+(1-(u(2)<3.5))*(u(4))))))))+((((u(2)<1.5)*(psi_r_rated)+(1-(u(2)<1.5))*(((u(2)<2.5)*(psi_fixed)+(1-(u(2)<2.5))*(((u(2)<3.5)*(u(3))+(1-(u(2)<3.5))*(u(4))))))))<=(psi_min))*(psi_min)))>=(psi_r_rated))*(psi_r_rated))))
  psi_target in : Mux
  trans_t : Fcn  Expr=(((((((abs(u(1))>trans_dw)+(abs(u(2)-u(3))>trans_dT))>0)*(trans_hold)+(1-(((abs(u(1))>trans_dw)+(abs(u(2)-u(3))>trans_dT))>0))*(u(4)))-Ts)>(0))*(((((abs(u(1))>trans_dw)+(abs(u(2)-u(3))>trans_dT))>0)*(trans_hold)+(1-(((abs(u(1))>trans_dw)+(abs(u(2)-u(3))>trans_dT))>0))*(u(4)))-Ts)+((((((abs(u(1))>trans_dw)+(abs(u(2)-u(3))>trans_dT))>0)*(trans_hold)+(1-(((abs(u(1))>trans_dw)+(abs(u(2)-u(3))>trans_dT))>0))*(u(4)))-Ts)<=(0))*(0))
  trans_t in : Mux
  trans_t(k-1) : UnitDelay  SampleTime=Ts  HasFrameUpgradeWarning=on
  psi_ref out : Outport
  dpsi_rate out : Outport  Port=2
  psi_ref_p out : Outport  Port=3
  trans_t_p out : Outport  Port=4
  dpsi_rate_p out : Outport  Port=5
  wires:
  e_w/1 -> trans_t in/1
  Te_ref/1 -> trans_t in/2, Te_ref_f in/2
  Te_ref_f(k-1)/1 -> trans_t in/3, Te_ref_f in/1
  trans_t(k-1)/1 -> trans_t in/4, trans_t_p out/1
  trans_t in/1 -> trans_t/1
  trans_t/1 -> trans_t(k-1)/1, psi_target in/1
  Te_ref_f in/1 -> Te_ref_f/1
  Te_ref_f/1 -> Te_ref_f(k-1)/1, abs Te_ref_f/1
  w_u/1 -> abs w_u/1
  abs w_u/1 -> LUT analytic/1, LUT ML/1, MLP network/1(w)
  abs Te_ref_f/1 -> LUT analytic/2, LUT ML/2, MLP network/2(T)
  lut_sel/1 -> LUT select/1
  LUT analytic/1 -> LUT select/2
  LUT ML/1 -> LUT select/3
  flux_sel/1 -> psi_target in/2
  LUT select/1 -> psi_target in/3
  MLP network/1(psi out) -> psi_target in/4
  psi_target in/1 -> psi_target/1
  psi_target/1 -> dpsi in/1
  psi_ref(k-1)/1 -> dpsi in/2, psi_ref in/1, psi_ref_p out/1
  dpsi in/1 -> dpsi/1
  dpsi/1 -> psi_ref in/2, dpsi_rate/1
  psi_ref in/1 -> psi_ref/1
  psi_ref/1 -> psi_ref(k-1)/1, psi_ref out/1
  dpsi_rate/1 -> dpsi_rate(k-1)/1, dpsi_rate out/1
  dpsi_rate(k-1)/1 -> dpsi_rate_p out/1

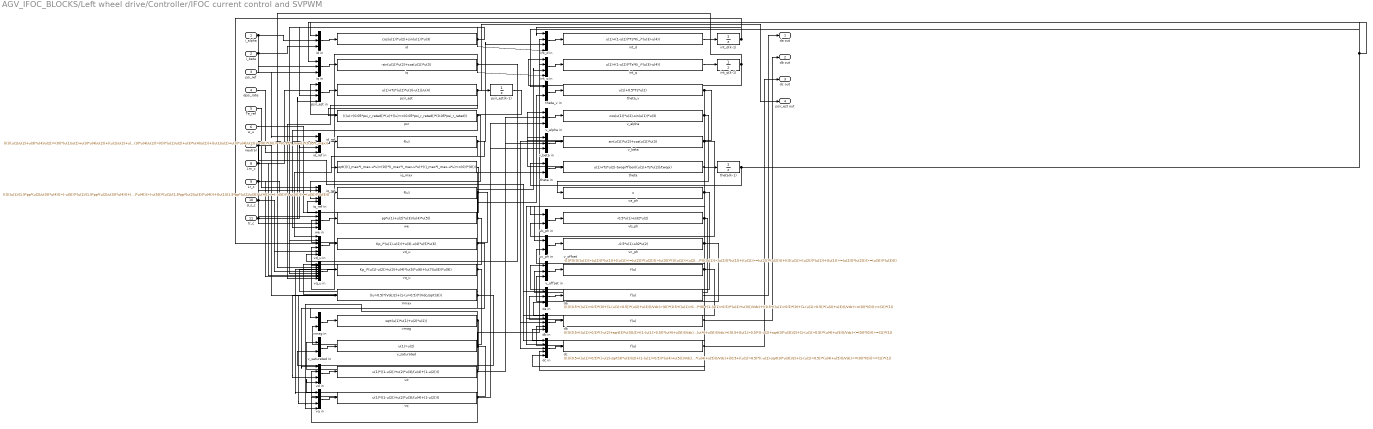
== system AGV_IFOC_BLOCKS/Left wheel drive/Controller/IFOC current control and SVPWM ==
  i_alpha : Inport
  i_beta : Inport  Port=2
  psi_ref : Inport  Port=3
  dpsi_rate : Inport  Port=4
  Te_ref : Inport  Port=5
  w_u : Inport  Port=6
  neutral : Inport  Port=7
  Lm_c : Inport  Port=8
  Lr_c : Inport  Port=9
  sLs_c : Inport  Port=10
  tr_c : Inport  Port=11
  Vmax : Fcn  Expr=((u>0.5)*(Vdc/2)+(1-(u>0.5))*(Vdc/sqrt(3)))
  da : Fcn  Expr=((((((0.5+((u(1)>0.5)*(0)+(1-(u(1)>0.5))*(u(2)+u(3)))/Vdc)>(0))*(0.5+((u(1)>0.5)*(0)+(1-(u(1)>0.5))*(u(2)+u(3)))/Vdc)+((0.5+((u(1)>0.5)*(0)+(1-(u(1)>0.5))*(u(2)+u(3)))/Vdc)<=(0))*(0)))<(1))*((((0.5+((u(1)>0.5)*(0)+(1-(u(1)>0.5))*(u(2)+u(3)))/Vdc)>(0))*(0.5+((u(1)>0.5)*(0)+(1-(u(1)>0.5))*(u(2)+u(3)))/Vdc)+((0.5+((u(1)>0.5)*(0)+(1-(u(1)>0.5))*(u(2)+u(3)))/Vdc)<=(0))*(0)))+(((((0.5+((u(1)>0.5)*(0)+(1-(u(1)>0.5))*(u(2)+u(3)))/Vdc)>(0))*(0.5+((u(1)>0.5)*(0)+(1-(u(1)>0.5))*(u(2)+u(3)))/Vdc)+((0.5+((u(1)>0.5)*(0)+(1-(u(1)>0.5))*(u(2)+u(3)))/Vdc)<=(0))*(0)))>=(1))*(1))
  da in : Mux  Inputs=3
  db : Fcn  Expr=((((((0.5+((u(1)>0.5)*((-u(2)+sqrt(3)*u(3))/2)+(1-(u(1)>0.5))*(u(4)+u(5)))/Vdc)>(0))*(0.5+((u(1)>0.5)*((-u(2)+sqrt(3)*u(3))/2)+(1-(u(1)>0.5))*(u(4)+u(5)))/Vdc)+((0.5+((u(1)>0.5)*((-u(2)+sqrt(3)*u(3))/2)+(1-(u(1)>0.5))*(u(4)+u(5)))/Vdc)<=(0))*(0)))<(1))*((((0.5+((u(1)>0.5)*((-u(2)+sqrt(3)*u(3))/2)+(1-(u(1)>0.5))*(u(4)+u(5)))/Vdc)>(0))*(0.5+((u(1)>0.5)*((-u(2)+sqrt(3)*u(3))/2)+(1-(u(1)>0.5))*(u(4)+u(5)))/Vdc)+((0.5+((u(1)>0.5)*((-u(2)+sqrt(3)*u(3))/2)+(1-(u(1)>0.5))*(u(4)+u(5)))/Vdc)<=(0))*(0)))+(((((0.5+((u(1)>0.5)*((-u(2)+sqrt(3)*u(3))/2)+(1-(u(1)>0.5))*(u(4)+u(5)))/Vdc)>(0))*(0.5+((u(1)>0.5)*((-u(2)+sqrt(3)*u(3))/2)+(1-(u(1)>0.5))*(u(4)+u(5)))/Vdc)+((0.5+((u(1)>0.5)*((-u(2)+sqrt(3)*u(3))/2)+(1-(u(1)>0.5))*(u(4)+u(5)))/Vdc)<=(0))*(0)))>=(1))*(1))
  db in : Mux  Inputs=5
  dc : Fcn  Expr=((((((0.5+((u(1)>0.5)*((-u(2)-sqrt(3)*u(3))/2)+(1-(u(1)>0.5))*(u(4)+u(5)))/Vdc)>(0))*(0.5+((u(1)>0.5)*((-u(2)-sqrt(3)*u(3))/2)+(1-(u(1)>0.5))*(u(4)+u(5)))/Vdc)+((0.5+((u(1)>0.5)*((-u(2)-sqrt(3)*u(3))/2)+(1-(u(1)>0.5))*(u(4)+u(5)))/Vdc)<=(0))*(0)))<(1))*((((0.5+((u(1)>0.5)*((-u(2)-sqrt(3)*u(3))/2)+(1-(u(1)>0.5))*(u(4)+u(5)))/Vdc)>(0))*(0.5+((u(1)>0.5)*((-u(2)-sqrt(3)*u(3))/2)+(1-(u(1)>0.5))*(u(4)+u(5)))/Vdc)+((0.5+((u(1)>0.5)*((-u(2)-sqrt(3)*u(3))/2)+(1-(u(1)>0.5))*(u(4)+u(5)))/Vdc)<=(0))*(0)))+(((((0.5+((u(1)>0.5)*((-u(2)-sqrt(3)*u(3))/2)+(1-(u(1)>0.5))*(u(4)+u(5)))/Vdc)>(0))*(0.5+((u(1)>0.5)*((-u(2)-sqrt(3)*u(3))/2)+(1-(u(1)>0.5))*(u(4)+u(5)))/Vdc)+((0.5+((u(1)>0.5)*((-u(2)-sqrt(3)*u(3))/2)+(1-(u(1)>0.5))*(u(4)+u(5)))/Vdc)<=(0))*(0)))>=(1))*(1))
  dc in : Mux  Inputs=5
  id : Fcn  Expr=cos(u(1))*u(2)+sin(u(1))*u(3)
  id in : Mux  Inputs=3
  id_ref : Fcn  Expr=((((((u(1)/u(2)+u(3)*u(4)/u(2))>(0))*(u(1)/u(2)+u(3)*u(4)/u(2))+((u(1)/u(2)+u(3)*u(4)/u(2))<=(0))*(0)))<(0.95*I_max))*((((u(1)/u(2)+u(3)*u(4)/u(2))>(0))*(u(1)/u(2)+u(3)*u(4)/u(2))+((u(1)/u(2)+u(3)*u(4)/u(2))<=(0))*(0)))+(((((u(1)/u(2)+u(3)*u(4)/u(2))>(0))*(u(1)/u(2)+u(3)*u(4)/u(2))+((u(1)/u(2)+u(3)*u(4)/u(2))<=(0))*(0)))>=(0.95*I_max))*(0.95*I_max))
  id_ref in : Mux
  int_d : Fcn  Expr=u(1)+(1-u(2))*Ts*Ki_i*(u(3)-u(4))
  int_d in : Mux
  int_d(k-1) : UnitDelay  SampleTime=Ts  HasFrameUpgradeWarning=on
  int_q : Fcn  Expr=u(1)+(1-u(2))*Ts*Ki_i*(u(3)-u(4))
  int_q in : Mux
  int_q(k-1) : UnitDelay  SampleTime=Ts  HasFrameUpgradeWarning=on
  iq : Fcn  Expr=-sin(u(1))*u(2)+cos(u(1))*u(3)
  iq in : Mux  Inputs=3
  iq_max : Fcn  Expr=sqrt((((I_max*I_max-u*u)>(0))*(I_max*I_max-u*u)+((I_max*I_max-u*u)<=(0))*(0)))
  iq_ref : Fcn  Expr=((((((u(1)/(1.5*pp*(u(2)/u(3))*u(4)))>(-u(5)))*(u(1)/(1.5*pp*(u(2)/u(3))*u(4)))+((u(1)/(1.5*pp*(u(2)/u(3))*u(4)))<=(-u(5)))*(-u(5))))<(u(5)))*((((u(1)/(1.5*pp*(u(2)/u(3))*u(4)))>(-u(5)))*(u(1)/(1.5*pp*(u(2)/u(3))*u(4)))+((u(1)/(1.5*pp*(u(2)/u(3))*u(4)))<=(-u(5)))*(-u(5))))+(((((u(1)/(1.5*pp*(u(2)/u(3))*u(4)))>(-u(5)))*(u(1)/(1.5*pp*(u(2)/u(3))*u(4)))+((u(1)/(1.5*pp*(u(2)/u(3))*u(4)))<=(-u(5)))*(-u(5))))>=(u(5)))*(u(5)))
  iq_ref in : Mux  Inputs=5
  psir_est : Fcn  Expr=u(1)+Ts*(u(2)*u(3)-u(1))/u(4)
  psir_est in : Mux
  psir_est(k-1) : UnitDelay  SampleTime=Ts  HasFrameUpgradeWarning=on
  psr : Fcn  Expr=(((u)>(0.05*psi_r_rated))*(u)+((u)<=(0.05*psi_r_rated))*(0.05*psi_r_rated))
  theta : Fcn  Expr=u(1)+Ts*u(2)-twopi*floor((u(1)+Ts*u(2))/twopi)
  theta in : Mux  Inputs=2
  theta(k-1) : UnitDelay  SampleTime=Ts  HasFrameUpgradeWarning=on
  theta_v : Fcn  Expr=u(1)+0.5*Ts*u(2)
  theta_v in : Mux  Inputs=2
  v_alpha : Fcn  Expr=cos(u(1))*u(2)-sin(u(1))*u(3)
  v_alpha in : Mux  Inputs=3
  v_beta : Fcn  Expr=sin(u(1))*u(2)+cos(u(1))*u(3)
  v_beta in : Mux  Inputs=3
  v_offset : Fcn  Expr=-0.5*(((((((u(1))>(u(2)))*(u(1))+((u(1))<=(u(2)))*(u(2))))>(u(3)))*((((u(1))>(u(2)))*(u(1))+((u(1))<=(u(2)))*(u(2))))+(((((u(1))>(u(2)))*(u(1))+((u(1))<=(u(2)))*(u(2))))<=(u(3)))*(u(3)))+((((((u(1))<(u(2)))*(u(1))+((u(1))>=(u(2)))*(u(2))))<(u(3)))*((((u(1))<(u(2)))*(u(1))+((u(1))>=(u(2)))*(u(2))))+(((((u(1))<(u(2)))*(u(1))+((u(1))>=(u(2)))*(u(2))))>=(u(3)))*(u(3))))
  v_offset in : Mux  Inputs=3
  v_saturated : Fcn  Expr=u(1)>u(2)
  v_saturated in : Mux  Inputs=2
  va_ph : Fcn  Expr=u
  vb_ph : Fcn  Expr=-0.5*u(1)+s32*u(2)
  vb_ph in : Mux  Inputs=2
  vc_ph : Fcn  Expr=-0.5*u(1)-s32*u(2)
  vc_ph in : Mux  Inputs=2
  vd : Fcn  Expr=u(1)*((1-u(2))+u(2)*u(3)/(u(4)+(1-u(2))))
  vd in : Mux
  vd_u : Fcn  Expr=Kp_i*(u(1)-u(2))+u(3)-u(4)*u(5)*u(6)
  vd_u in : Mux  Inputs=6
  vmag : Fcn  Expr=sqrt(u(1)*u(1)+u(2)*u(2))
  vmag in : Mux  Inputs=2
  vq : Fcn  Expr=u(1)*((1-u(2))+u(2)*u(3)/(u(4)+(1-u(2))))
  vq in : Mux
  vq_u : Fcn  Expr=Kp_i*(u(1)-u(2))+u(3)+u(4)*(u(5)*u(6)+(u(7)/u(8))*u(9))
  vq_u in : Mux  Inputs=9
  we : Fcn  Expr=pp*u(1)+u(2)*u(3)/(u(4)*u(5))
  we in : Mux  Inputs=5
  da out : Outport
  db out : Outport  Port=2
  dc out : Outport  Port=3
  psir_est out : Outport  Port=4
  wires:
  theta(k-1)/1 -> id in/1, iq in/1, theta_v in/1, theta in/1
  i_alpha/1 -> id in/2, iq in/2
  i_beta/1 -> id in/3, iq in/3
  id in/1 -> id/1
  iq in/1 -> iq/1
  psir_est(k-1)/1 -> psir_est in/1
  Lm_c/1 -> psir_est in/2, id_ref in/2, iq_ref in/2, we in/2, vq_u in/7
  id/1 -> psir_est in/3, vd_u in/2, vq_u in/6, int_d in/4
  tr_c/1 -> psir_est in/4, id_ref in/3, we in/4
  psir_est in/1 -> psir_est/1
  psir_est/1 -> psir_est(k-1)/1, psr/1, vq_u in/9, psir_est out/1
  psi_ref/1 -> id_ref in/1
  dpsi_rate/1 -> id_ref in/4
  id_ref in/1 -> id_ref/1
  id_ref/1 -> iq_max/1, vd_u in/1, int_d in/3
  Te_ref/1 -> iq_ref in/1
  Lr_c/1 -> iq_ref in/3, vq_u in/8
  psr/1 -> iq_ref in/4, we in/5
  iq_max/1 -> iq_ref in/5
  iq_ref in/1 -> iq_ref/1
  w_u/1 -> we in/1
  iq_ref/1 -> we in/3, vq_u in/1, int_q in/3
  we in/1 -> we/1
  int_d(k-1)/1 -> vd_u in/3, int_d in/1
  we/1 -> vd_u in/4, vq_u in/4, theta_v in/2, theta in/2
  sLs_c/1 -> vd_u in/5, vq_u in/5
  iq/1 -> vd_u in/6, vq_u in/2, int_q in/4
  vd_u in/1 -> vd_u/1
  int_q(k-1)/1 -> vq_u in/3, int_q in/1
  vq_u in/1 -> vq_u/1
  neutral/1 -> Vmax/1, da in/1, db in/1, dc in/1
  vd_u/1 -> vmag in/1, vd in/1
  vq_u/1 -> vmag in/2, vq in/1
  vmag in/1 -> vmag/1
  vmag/1 -> v_saturated in/1, vd in/4, vq in/4
  Vmax/1 -> v_saturated in/2, vd in/3, vq in/3
  v_saturated in/1 -> v_saturated/1
  v_saturated/1 -> vd in/2, vq in/2, int_d in/2, int_q in/2
  vd in/1 -> vd/1
  vq in/1 -> vq/1
  int_d in/1 -> int_d/1
  int_d/1 -> int_d(k-1)/1
  int_q in/1 -> int_q/1
  int_q/1 -> int_q(k-1)/1
  theta_v in/1 -> theta_v/1
  theta_v/1 -> v_alpha in/1, v_beta in/1
  vd/1 -> v_alpha in/2, v_beta in/2
  vq/1 -> v_alpha in/3, v_beta in/3
  v_alpha in/1 -> v_alpha/1
  v_beta in/1 -> v_beta/1
  theta in/1 -> theta/1
  theta/1 -> theta(k-1)/1
  v_alpha/1 -> va_ph/1, vb_ph in/1, vc_ph in/1, db in/2, dc in/2
  v_beta/1 -> vb_ph in/2, vc_ph in/2, db in/3, dc in/3
  vb_ph in/1 -> vb_ph/1
  vc_ph in/1 -> vc_ph/1
  va_ph/1 -> v_offset in/1, da in/2
  vb_ph/1 -> v_offset in/2, db in/4
  vc_ph/1 -> v_offset in/3, dc in/4
  v_offset in/1 -> v_offset/1
  v_offset/1 -> da in/3, db in/5, dc in/5
  da in/1 -> da/1
  db in/1 -> db/1
  dc in/1 -> dc/1
  da/1 -> da out/1
  db/1 -> db out/1
  dc/1 -> dc out/1

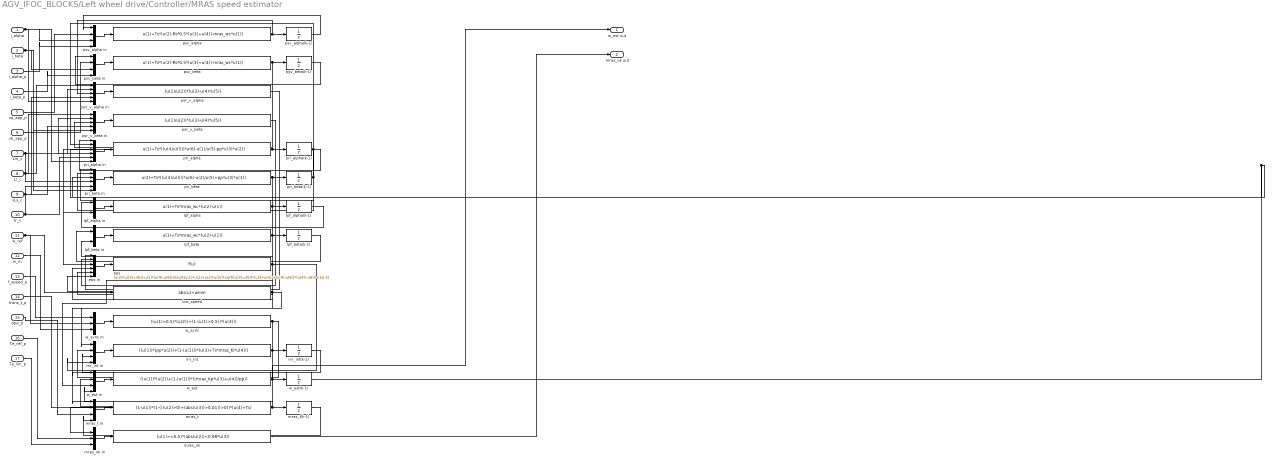
== system AGV_IFOC_BLOCKS/Left wheel drive/Controller/MRAS speed estimator ==
  i_alpha : Inport
  i_beta : Inport  Port=2
  i_alpha_p : Inport  Port=3
  i_beta_p : Inport  Port=4
  va_app_p : Inport  Port=5
  vb_app_p : Inport  Port=6
  Lm_c : Inport  Port=7
  Lr_c : Inport  Port=8
  sLs_c : Inport  Port=9
  tr_c : Inport  Port=10
  w_ref : Inport  Port=11
  w_m : Inport  Port=12
  f_speed_p : Inport  Port=13
  trans_t_p : Inport  Port=14
  dpsi_p : Inport  Port=15
  Te_ref_p : Inport  Port=16
  Te_lim_p : Inport  Port=17
  eps : Fcn  Expr=(u(2)*(u(3)-u(5))-u(1)*(u(4)-u(6)))/(sqrt(u(1)*u(1)+u(2)*u(2))*sqrt((u(3)-u(5))*(u(3)-u(5))+(u(4)-u(6))*(u(4)-u(6)))+1e-3)
  eps in : Mux  Inputs=6
  low_speed : Fcn  Expr=abs(u)<wmin
  lpf_alpha : Fcn  Expr=u(1)+Ts*mras_wc*(u(2)-u(1))
  lpf_alpha in : Mux  Inputs=2
  lpf_alpha(k-1) : UnitDelay  SampleTime=Ts  HasFrameUpgradeWarning=on
  lpf_beta : Fcn  Expr=u(1)+Ts*mras_wc*(u(2)-u(1))
  lpf_beta in : Mux  Inputs=2
  lpf_beta(k-1) : UnitDelay  SampleTime=Ts  HasFrameUpgradeWarning=on
  mr_int : Fcn  Expr=((u(1))*(pp*u(2))+(1-(u(1)))*(u(3)+Ts*mras_Ki*u(4)))
  mr_int in : Mux
  mr_int(k-1) : UnitDelay  SampleTime=Ts  HasFrameUpgradeWarning=on
  mras_ok : Fcn  Expr=(u(1)>=0.5)*(abs(u(2))<0.98*u(3))
  mras_ok in : Mux  Inputs=3
  mras_t : Fcn  Expr=(1-u(1))*(1-(((u(2)>0)+(abs(u(3))>0.01))>0))*(u(4)+Ts)
  mras_t in : Mux
  mras_t(k-1) : UnitDelay  SampleTime=Ts  HasFrameUpgradeWarning=on
  pri_alpha : Fcn  Expr=u(1)+Ts*((u(4)/u(5))*u(6)-u(1)/u(5)-pp*u(3)*u(2))
  pri_alpha in : Mux  Inputs=6
  pri_alpha(k-1) : UnitDelay  SampleTime=Ts  HasFrameUpgradeWarning=on
  pri_beta : Fcn  Expr=u(2)+Ts*((u(4)/u(5))*u(6)-u(2)/u(5)+pp*u(3)*u(1))
  pri_beta in : Mux  Inputs=6
  pri_beta(k-1) : UnitDelay  SampleTime=Ts  HasFrameUpgradeWarning=on
  psr_v_alpha : Fcn  Expr=(u(1)/u(2))*(u(3)-u(4)*u(5))
  psr_v_alpha in : Mux  Inputs=5
  psr_v_beta : Fcn  Expr=(u(1)/u(2))*(u(3)-u(4)*u(5))
  psr_v_beta in : Mux  Inputs=5
  psv_alpha : Fcn  Expr=u(1)+Ts*(u(2)-Rs*0.5*(u(3)+u(4))-mras_wc*u(1))
  psv_alpha in : Mux
  psv_alpha(k-1) : UnitDelay  SampleTime=Ts  HasFrameUpgradeWarning=on
  psv_beta : Fcn  Expr=u(1)+Ts*(u(2)-Rs*0.5*(u(3)+u(4))-mras_wc*u(1))
  psv_beta in : Mux
  psv_beta(k-1) : UnitDelay  SampleTime=Ts  HasFrameUpgradeWarning=on
  w_est : Fcn  Expr=((u(1))*(u(2))+(1-(u(1)))*((mras_Kp*u(3)+u(4))/pp))
  w_est in : Mux
  w_est(k-1) : UnitDelay  SampleTime=Ts  HasFrameUpgradeWarning=on
  w_sync : Fcn  Expr=((u(1)>0.5)*(u(2))+(1-(u(1)>0.5))*(u(3)))
  w_sync in : Mux  Inputs=3
  w_est out : Outport
  mras_ok out : Outport  Port=2
  wires:
  psv_alpha(k-1)/1 -> psv_alpha in/1
  va_app_p/1 -> psv_alpha in/2
  i_alpha/1 -> psv_alpha in/3, psr_v_alpha in/5, pri_alpha in/6
  i_alpha_p/1 -> psv_alpha in/4
  psv_alpha in/1 -> psv_alpha/1
  psv_alpha/1 -> psv_alpha(k-1)/1, psr_v_alpha in/3
  psv_beta(k-1)/1 -> psv_beta in/1
  vb_app_p/1 -> psv_beta in/2
  i_beta/1 -> psv_beta in/3, psr_v_beta in/5, pri_beta in/6
  i_beta_p/1 -> psv_beta in/4
  psv_beta in/1 -> psv_beta/1
  psv_beta/1 -> psv_beta(k-1)/1, psr_v_beta in/3
  Lr_c/1 -> psr_v_alpha in/1, psr_v_beta in/1
  Lm_c/1 -> psr_v_alpha in/2, psr_v_beta in/2, pri_alpha in/4, pri_beta in/4
  sLs_c/1 -> psr_v_alpha in/4, psr_v_beta in/4
  psr_v_alpha in/1 -> psr_v_alpha/1
  psr_v_beta in/1 -> psr_v_beta/1
  pri_alpha(k-1)/1 -> pri_alpha in/1, pri_beta in/1
  pri_beta(k-1)/1 -> pri_alpha in/2, pri_beta in/2
  w_est(k-1)/1 -> pri_alpha in/3, pri_beta in/3
  tr_c/1 -> pri_alpha in/5, pri_beta in/5
  pri_alpha in/1 -> pri_alpha/1
  pri_alpha/1 -> pri_alpha(k-1)/1, lpf_alpha in/2, eps in/3
  pri_beta in/1 -> pri_beta/1
  pri_beta/1 -> pri_beta(k-1)/1, lpf_beta in/2, eps in/4
  lpf_alpha(k-1)/1 -> lpf_alpha in/1
  lpf_alpha in/1 -> lpf_alpha/1
  lpf_alpha/1 -> lpf_alpha(k-1)/1, eps in/5
  lpf_beta(k-1)/1 -> lpf_beta in/1
  lpf_beta in/1 -> lpf_beta/1
  lpf_beta/1 -> lpf_beta(k-1)/1, eps in/6
  psr_v_alpha/1 -> eps in/1
  psr_v_beta/1 -> eps in/2
  eps in/1 -> eps/1
  w_ref/1 -> low_speed/1, w_sync in/2
  f_speed_p/1 -> w_sync in/1
  w_m/1 -> w_sync in/3
  w_sync in/1 -> w_sync/1
  low_speed/1 -> mr_int in/1, w_est in/1, mras_t in/1
  w_sync/1 -> mr_int in/2, w_est in/2
  mr_int(k-1)/1 -> mr_int in/3
  eps/1 -> mr_int in/4, w_est in/3
  mr_int in/1 -> mr_int/1
  mr_int/1 -> mr_int(k-1)/1, w_est in/4
  w_est in/1 -> w_est/1
  w_est/1 -> w_est(k-1)/1, w_est out/1
  trans_t_p/1 -> mras_t in/2
  dpsi_p/1 -> mras_t in/3
  mras_t(k-1)/1 -> mras_t in/4
  mras_t in/1 -> mras_t/1
  mras_t/1 -> mras_t(k-1)/1, mras_ok in/1
  Te_ref_p/1 -> mras_ok in/2
  Te_lim_p/1 -> mras_ok in/3
  mras_ok in/1 -> mras_ok/1
  mras_ok/1 -> mras_ok out/1

== system AGV_IFOC_BLOCKS/Left wheel drive/Controller/Model inductances ==
  psi_ref_p : Inport
  D_c : Fcn  Expr=u(2)*u(3)-u(1)*u(1)
  D_c in : Mux  Inputs=3
  Lm_c : Fcn  Expr=Lm_rated+ctrl_sat*(Lm0/(1+sat_a*((((u)>(0.05))*(u)+((u)<=(0.05))*(0.05))/psi_k)^sat_b)-Lm_rated)
  Lr_c : Fcn  Expr=Llr+u
  Ls_c : Fcn  Expr=Lls+u
  sLs_c : Fcn  Expr=u(2)-u(1)*u(1)/u(3)
  sLs_c in : Mux  Inputs=3
  tr_c : Fcn  Expr=u/Rr
  Lm_c out : Outport
  Ls_c out : Outport  Port=2
  Lr_c out : Outport  Port=3
  sLs_c out : Outport  Port=4
  tr_c out : Outport  Port=5
  D_c out : Outport  Port=6
  wires:
  psi_ref_p/1 -> Lm_c/1
  Lm_c/1 -> Ls_c/1, Lr_c/1, sLs_c in/1, D_c in/1, Lm_c out/1
  Ls_c/1 -> sLs_c in/2, D_c in/2, Ls_c out/1
  Lr_c/1 -> sLs_c in/3, tr_c/1, D_c in/3, Lr_c out/1
  sLs_c in/1 -> sLs_c/1
  D_c in/1 -> D_c/1
  sLs_c/1 -> sLs_c out/1
  tr_c/1 -> tr_c out/1
  D_c/1 -> D_c out/1

== system AGV_IFOC_BLOCKS/Left wheel drive/Controller/Speed controller ==
  w_ref : Inport
  w_u : Inport  Port=2
  Te_lim : Inport  Port=3
  mode : Inport  Port=4
  Te_pi : Fcn  Expr=((((((u(1))>(-u(2)))*(u(1))+((u(1))<=(-u(2)))*(-u(2))))<(u(2)))*((((u(1))>(-u(2)))*(u(1))+((u(1))<=(-u(2)))*(-u(2))))+(((((u(1))>(-u(2)))*(u(1))+((u(1))<=(-u(2)))*(-u(2))))>=(u(2)))*(u(2)))
  Te_pi in : Mux  Inputs=2
  Te_ref : Fcn  Expr=((u(1)>1.5)*(relay_bias+u(2)*relay_T)+(1-(u(1)>1.5))*(u(3)))
  Te_ref in : Mux  Inputs=3
  Te_ref(k-1) : UnitDelay  SampleTime=Ts  HasFrameUpgradeWarning=on
  Te_u : Fcn  Expr=Kp_w*u(1)+u(2)
  Te_u in : Mux  Inputs=2
  e_w : Fcn  Expr=u(1)-u(2)
  e_w in : Mux  Inputs=2
  int_w : Fcn  Expr=((u(1)>1.5)*(u(2))+(1-(u(1)>1.5))*(((((abs(u(3))<=u(4))+(abs(((u(5)>0)-(u(5)<0))-((u(3)>0)-(u(3)<0)))>0.5))>0)*(((((((u(2)+Ts*Ki_w*u(5))>(-u(4)))*(u(2)+Ts*Ki_w*u(5))+((u(2)+Ts*Ki_w*u(5))<=(-u(4)))*(-u(4))))<(u(4)))*((((u(2)+Ts*Ki_w*u(5))>(-u(4)))*(u(2)+Ts*Ki_w*u(5))+((u(2)+Ts*Ki_w*u(5))<=(-u(4)))*(-u(4))))+(((((u(2)+Ts*Ki_w*u(5))>(-u(4)))*(u(2)+Ts*Ki_w*u(5))+((u(2)+Ts*Ki_w*u(5))<=(-u(4)))*(-u(4))))>=(u(4)))*(u(4))))+(1-(((abs(u(3))<=u(4))+(abs(((u(5)>0)-(u(5)<0))-((u(3)>0)-(u(3)<0)))>0.5))>0))*(u(2)))))
  int_w in : Mux  Inputs=5
  int_w(k-1) : UnitDelay  SampleTime=Ts  HasFrameUpgradeWarning=on
  relay : Fcn  Expr=((u(1)>1.5)*(((u(2)>relay_h)*(1)+(1-(u(2)>relay_h))*(((u(2)<-relay_h)*(-1)+(1-(u(2)<-relay_h))*(u(3))))))+(1-(u(1)>1.5))*(u(3)))
  relay in : Mux  Inputs=3
  relay(k-1) : UnitDelay  InitialCondition=1  SampleTime=Ts  HasFrameUpgradeWarning=on
  Te_ref out : Outport
  e_w out : Outport  Port=2
  Te_ref_p out : Outport  Port=3
  wires:
  w_ref/1 -> e_w in/1
  w_u/1 -> e_w in/2
  e_w in/1 -> e_w/1
  mode/1 -> relay in/1, Te_ref in/1, int_w in/1
  e_w/1 -> relay in/2, Te_u in/1, int_w in/5, e_w out/1
  relay(k-1)/1 -> relay in/3
  relay in/1 -> relay/1
  relay/1 -> relay(k-1)/1, Te_ref in/2
  int_w(k-1)/1 -> Te_u in/2, int_w in/2
  Te_u in/1 -> Te_u/1
  Te_u/1 -> Te_pi in/1, int_w in/3
  Te_lim/1 -> Te_pi in/2, int_w in/4
  Te_pi in/1 -> Te_pi/1
  Te_pi/1 -> Te_ref in/3
  Te_ref in/1 -> Te_ref/1
  Te_ref/1 -> Te_ref(k-1)/1, Te_ref out/1
  int_w in/1 -> int_w/1
  int_w/1 -> int_w(k-1)/1
  Te_ref(k-1)/1 -> Te_ref_p out/1

== system AGV_IFOC_BLOCKS/Left wheel drive/Inverter and motor/Core loss ==
  psim_alpha : Inport
  psim_beta : Inport  Port=2
  Pfe : Fcn  Expr=(kh*abs(u(1))+ke*u(1)*u(1))*(u(2)*u(2)+u(3)*u(3))
  Pfe in : Mux  Inputs=3
  angle step : Fcn  Expr=u(1)-u(2)
  angle step in : Mux  Inputs=2
  fe : Fcn  Expr=(u-twopi*floor(u/twopi+0.5))/(twopi*Ts)
  flux angle : Fcn  Expr=atan2(u(2),u(1))
  flux angle in : Mux  Inputs=2
  flux angle(k-1) : UnitDelay  SampleTime=Ts  HasFrameUpgradeWarning=on
  psim_alpha sample : ZeroOrderHold  SampleTime=Ts
  psim_beta sample : ZeroOrderHold  SampleTime=Ts
  Pfe out : Outport
  wires:
  psim_alpha/1 -> psim_alpha sample/1
  psim_beta/1 -> psim_beta sample/1
  psim_alpha sample/1 -> flux angle in/1, Pfe in/2
  psim_beta sample/1 -> flux angle in/2, Pfe in/3
  flux angle in/1 -> flux angle/1
  flux angle/1 -> flux angle(k-1)/1, angle step in/1
  flux angle(k-1)/1 -> angle step in/2
  angle step in/1 -> angle step/1
  angle step/1 -> fe/1
  fe/1 -> Pfe in/1
  Pfe in/1 -> Pfe/1
  Pfe/1 -> Pfe out/1
